simulink model "course_lab5_bandwidth"  (R2024b)
settings: Solver=ode45  StartTime=0.0  StopTime=0.0001  MaxStep=6.666666666666667e-08  RelTol=1e-7  AbsTol=1e-9
model workspace (MAT data in the model file):
  A = 0.05
  GBW = 1000000
  K = 1
  T = 0.001
  den = [1.59154943092e-07 1]
  frequency = 100000
  num = [0 1]
  web_input = timeseries
  web_input.Name = 'unnamed'
  web_input.DataInfo = tsdata.datametadata
  web_input.DataInfo.Interpolation = tsdata.interpolation
  web_input.DataInfo.Interpolation.Fhandle : function handle (value not decoded)
  web_input.DataInfo.Interpolation.Name = 'linear'
  web_input.TimeInfo = tsdata.timemetadata
  web_input.TimeInfo.Length = 1501
  web_input.TimeInfo.DuplicateTimes = 0
  web_input.TimeInfo.Time_ = [0 6.66666666667e-08 1.33333333333e-07 2e-07 2.66666666667e-07 3.33333333333e-07 4e-07 4.66666666667e-07 5.33333333333e-07 6e-07 6.66666666667e-07 7.33333333333e-07 ... (1501 elements, 1501x1)]
  web_input.TimeInfo.Initialized = 1
  web_input.QualityInfo = tsdata.qualmetadata
  web_input.Data_ = [0 0.00209378268646 0.00418389216662 0.00626666167822 0.00833843733581 0.0103955845409 0.0124344943582 0.0144515898472 0.0164433323369 0.0184062276342 0.0203368321538 0.0222317589592 ... (1501 elements, 1501x1)]
  wn = 22.36068
  zeta = 0.223607
settings Model: Creator=33657  LastModifiedBy=33657

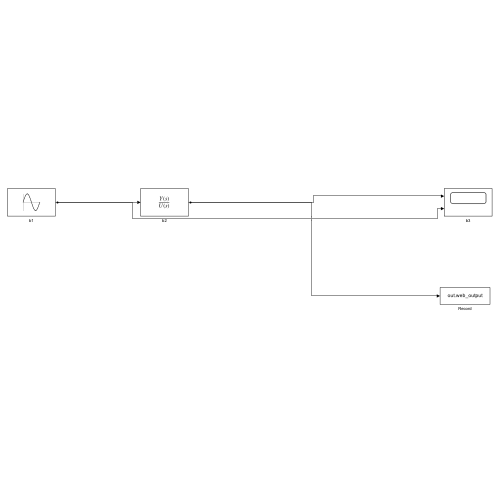
[thumbnail: Simulink's stored preview of the top-level diagram]
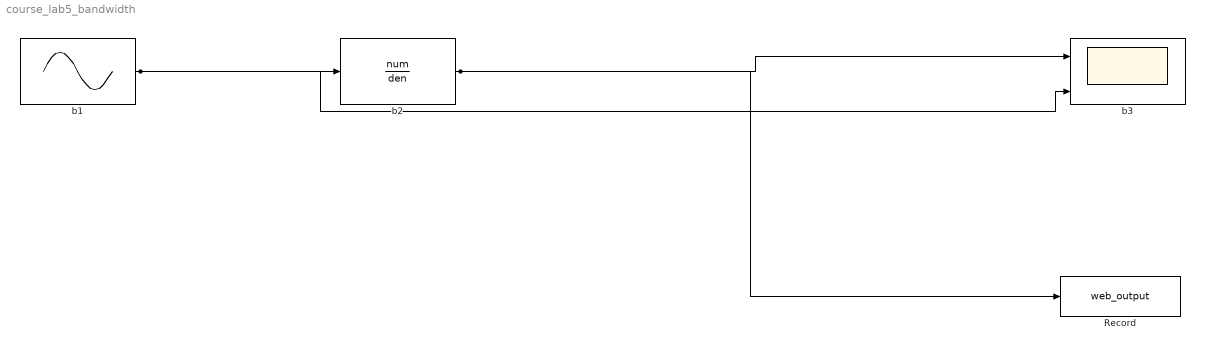
== system course_lab5_bandwidth ==
  Record : ToWorkspace  VariableName=web_output  SaveFormat=Timeseries  SampleTime=-1
  b1 : Sin  Amplitude=A  Frequency=2*pi*frequency  SampleTime=0
  b2 : TransferFcn  Numerator=num  Denominator=den
  b3 : Scope  NumInputPorts=2
  wires:
  b1/1 -> b2/1, b3/2
  b2/1 -> b3/1, Record/1
